simulink model "ele_t_cal"  (R2022b)
settings: Solver=VariableStepAuto  StartTime=0.0  StopTime=10.0  RelTol=1e-3
InitFcn:
  | flux = 2.0
settings Model: Creator=15403  LastModifiedBy=15403

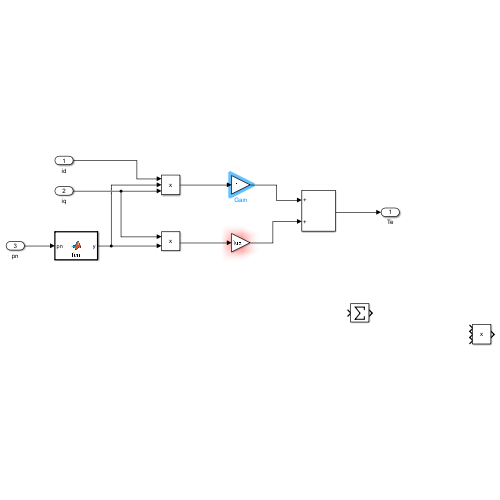
[thumbnail: Simulink's stored preview of the top-level diagram]
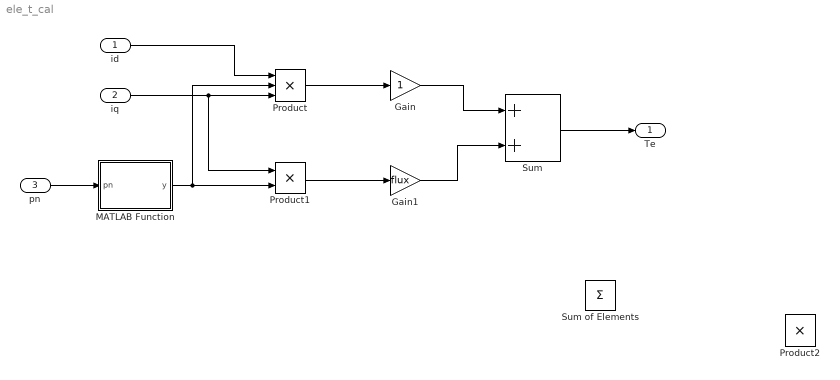
== system ele_t_cal ==
  id : Inport
  iq : Inport  Port=2
  pn : Inport  Port=3
  Gain : Gain
  Gain1 : Gain  Gain=flux
  MATLAB Function : MATLAB Function  TreatAsAtomicUnit=on
  Product : Product  Inputs=3
  Product1 : Product
  Product2 : Product  Inputs=3
  Sum : Sum
  Sum of Elements : Sum  Inputs=+
  Te : Outport
  wires:
  id/1 -> Product/1
  iq/1 -> Product1/1, Product/3
  pn/1 -> MATLAB Function/1(pn)
  MATLAB Function/1(y) -> Product/2, Product1/2
  Product1/1 -> Gain1/1
  Gain1/1 -> Sum/2
  Sum/1 -> Te/1
  Product/1 -> Gain/1
  Gain/1 -> Sum/1

== matlab function ele_t_cal/MATLAB Function ==
  data: pn input; y output
function y = fcn(pn)

y = pn * 3 / 2;
